simulink model "T_C"  (R2017b)
settings: Solver=VariableStepAuto  StartTime=0.0  StopTime=600  RelTol=1e-3
libraries: simulink x6, fuzblock x1, vrlib x1
settings Model: Creator=Hesam  LastModifiedBy=Hesam

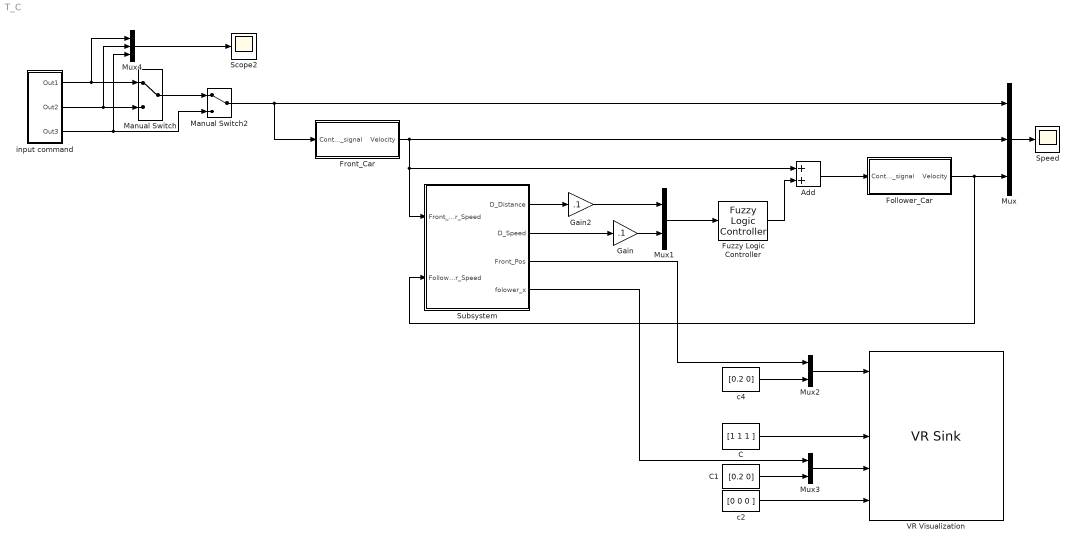
== system T_C ==
  Add : Sum
  C : Constant  Value=[1 1 1 ]
  C1 : Constant  Value=[0.2 0]
  Follower_Car : Subsystem
  Front_Car : Subsystem
  Fuzzy Logic Controller : fuzblock/Fuzzy Logic  Controller  FIS=Rule  OutputSampleNumber=101  DataType=double  FuzzifiedInputs=off  RuleFiringStrengths=off  RuleOutputs=off  AggregatedOutputs=off  SimulateUsing=Interpreted execution
  Gain : Gain  Gain=.1
  Gain2 : Gain  Gain=.1
  Manual Switch : ManualSwitch
  Manual Switch2 : ManualSwitch
  Mux : Mux  Inputs=3
  Mux1 : Mux  Inputs=2
  Mux2 : Mux  Inputs=2
  Mux3 : Mux  Inputs=2
  Mux4 : Mux  Inputs=3
  Scope2 : Scope
  "Speed " : Scope
  Subsystem : Subsystem
  VR Visualization : vrlib/VR Sink  InstantiateOnLoad=on  SampleTime=-1  ViewEnable=on  RemoteChange=off  RemoteView=off  FieldsWritten=Car_1.Car_Position.3.1.1.double#Car_1.SteeringWheel1_Rotation.4.1.1.double#Car_1.Car_DiffuseColor.3.1.1.double#Car_2.Car_Position.3.1.1.double#Car_2.Car_DiffuseColor.3.1.1.double  WorldFileName=octavia_scene_lchg_2cars.wrl  WorldDescription=Vehicle Dynamics Visualization - Multiple Vehicles  AutoView=on  VideoDimensions=[]  AllowVariableSize=off
      settings: SourceProductBaseCode=VR
  c2 : Constant  Value=[0 0 0 ]
  c4 : Constant  Value=[0.2 0]
  input command : Subsystem
  wires:
  Mux2/1 -> VR Visualization/1
  Add/1 -> Follower_Car/1(Controll_signal)
  Fuzzy Logic Controller/1 -> Add/2
  c2/1 -> VR Visualization/5
  Mux1/1 -> Fuzzy Logic Controller/1
  Mux3/1 -> VR Visualization/4
  C1/1 -> Mux3/2
  Gain/1 -> Mux1/2
  C/1 -> VR Visualization/3
  Gain2/1 -> Mux1/1
  Front_Car/1(Velocity) -> Subsystem/1("Front_Car_Speed "), Add/1, Mux/2
  Subsystem/2(D_Speed) -> Gain/1
  c4/1 -> Mux2/2
  Follower_Car/1(Velocity) -> Subsystem/2(Follower_Car_Speed), Mux/3
  Subsystem/3(Front_Pos) -> Mux2/1
  Subsystem/4(folower_x) -> Mux3/1
  Subsystem/1("D_Distance ") -> Gain2/1
  Mux/1 -> "Speed "/1
  Manual Switch/1 -> Manual Switch2/1
  input command/1(Out1) -> Mux4/1, Manual Switch/1
  input command/2(Out2) -> Manual Switch/2, Mux4/2
  Mux4/1 -> Scope2/1
  Manual Switch2/1 -> Front_Car/1("Control_signal "), Mux/1
  input command/3(Out3) -> Manual Switch2/2, Mux4/3

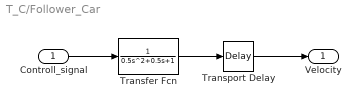
== system T_C/Follower_Car ==
  Controll_signal : Inport
  Transfer Fcn : TransferFcn  Denominator=[0.5 0.5 1]
  Transport Delay : TransportDelay  DelayTime=0.1
  Velocity : Outport
  wires:
  Controll_signal/1 -> Transfer Fcn/1
  Transfer Fcn/1 -> Transport Delay/1
  Transport Delay/1 -> Velocity/1

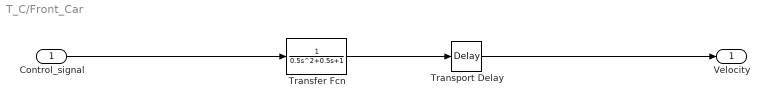
== system T_C/Front_Car ==
  "Control_signal " : Inport
  Transfer Fcn : TransferFcn  Denominator=[0.5 0.5 1]
  Transport Delay : TransportDelay  DelayTime=0.1
  Velocity : Outport
  wires:
  Transport Delay/1 -> Velocity/1
  Transfer Fcn/1 -> Transport Delay/1
  "Control_signal "/1 -> Transfer Fcn/1

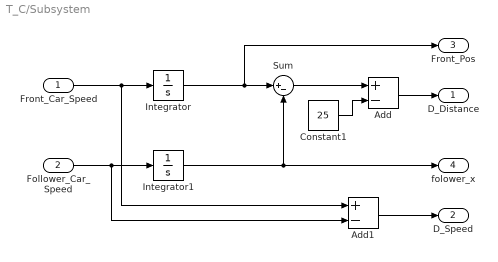
== system T_C/Subsystem ==
  "Front_Car_Speed " : Inport
  Follower_Car_Speed : Inport  Port=2
  Add : Sum  Inputs=+-
  Add1 : Sum  Inputs=+-
  Constant1 : Constant  Value=25
  Integrator : Integrator  InitialCondition=5
  Integrator1 : Integrator
  Sum : Sum  Inputs=|+-
  "D_Distance " : Outport
  D_Speed : Outport  Port=2
  Front_Pos : Outport  Port=3
  folower_x : Outport  Port=4
  wires:
  "Front_Car_Speed "/1 -> Add1/1, Integrator/1
  Follower_Car_Speed/1 -> Integrator1/1, Add1/2
  Sum/1 -> Add/1
  Constant1/1 -> Add/2
  Integrator1/1 -> Sum/2, folower_x/1
  Integrator/1 -> Front_Pos/1, Sum/1
  Add1/1 -> D_Speed/1
  Add/1 -> "D_Distance "/1

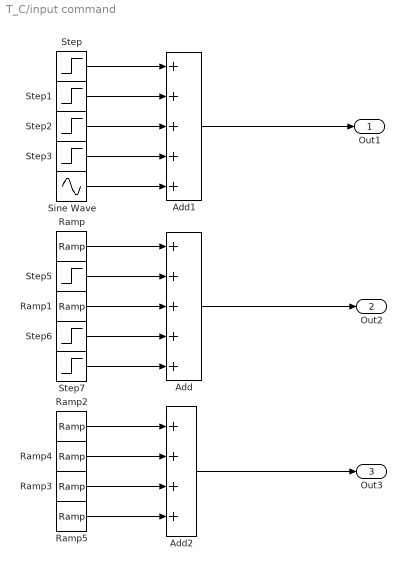
== system T_C/input command ==
  Add : Sum  Inputs=+++++
  Add1 : Sum  Inputs=+++++
  Add2 : Sum  Inputs=++++
  Ramp : simulink/Sources/Ramp  slope=1  start=0  X0=0
  Ramp1 : simulink/Sources/Ramp  slope=-1  start=200  X0=0
  Ramp2 : simulink/Sources/Ramp  slope=2  start=0  X0=0
  Ramp3 : simulink/Sources/Ramp  slope=-1  start=150  X0=0
  Ramp4 : simulink/Sources/Ramp  slope=-2  start=100  X0=0
  Ramp5 : simulink/Sources/Ramp  slope=1  start=200  X0=0
  Sine Wave : Sin  Amplitude=5  Frequency=0.1  SampleTime=0
  Step : Step  Time=0  After=30  SampleTime=0
  Step1 : Step  Time=100  After=20  SampleTime=0
  Step2 : Step  Time=200  After=-10  SampleTime=0
  Step3 : Step  Time=300  After=-5  SampleTime=0
  Step5 : Step  Time=100  After=10  SampleTime=0
  Step6 : Step  Time=300  After=-10  SampleTime=0
  Step7 : Step  Time=400  After=-20  SampleTime=0
  Out1 : Outport
  Out2 : Outport  Port=2
  Out3 : Outport  Port=3
  wires:
  Add1/1 -> Out1/1
  Ramp/1 -> Add/1
  Step5/1 -> Add/2
  Ramp1/1 -> Add/3
  Step6/1 -> Add/4
  Step7/1 -> Add/5
  Add/1 -> Out2/1
  Step3/1 -> Add1/4
  Step2/1 -> Add1/3
  Step1/1 -> Add1/2
  Step/1 -> Add1/1
  Sine Wave/1 -> Add1/5
  Ramp5/1 -> Add2/4
  Add2/1 -> Out3/1
  Ramp4/1 -> Add2/2
  Ramp2/1 -> Add2/1
  Ramp3/1 -> Add2/3
